simulink library "lib_SecCtrl_MASmsg"  (R2026a)
settings: Solver=VariableStepAuto
undefined symbols (not defined in the file): buses_lf, DiscIntNeverNeededParam, entity, iPs_lf, iQs_lf, last_send, m, Ps_lf, Qs_lf, set_DG_up, set_extra_satur, set_sending_cost, v_buses_mod
libraries: simulink x400, sl_discontinuities x10, eeGeneralControl x5
(part 1 of 12)
settings Model: Creator=atomas  LastModifiedBy=atomas

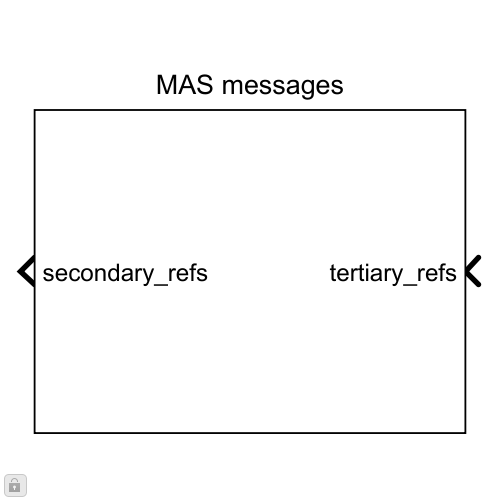
[thumbnail: Simulink's stored preview of the top-level diagram]
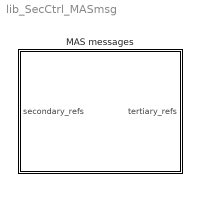
== system lib_SecCtrl_MASmsg ==
  MAS messages : Subsystem  VariantControl=MAS messages

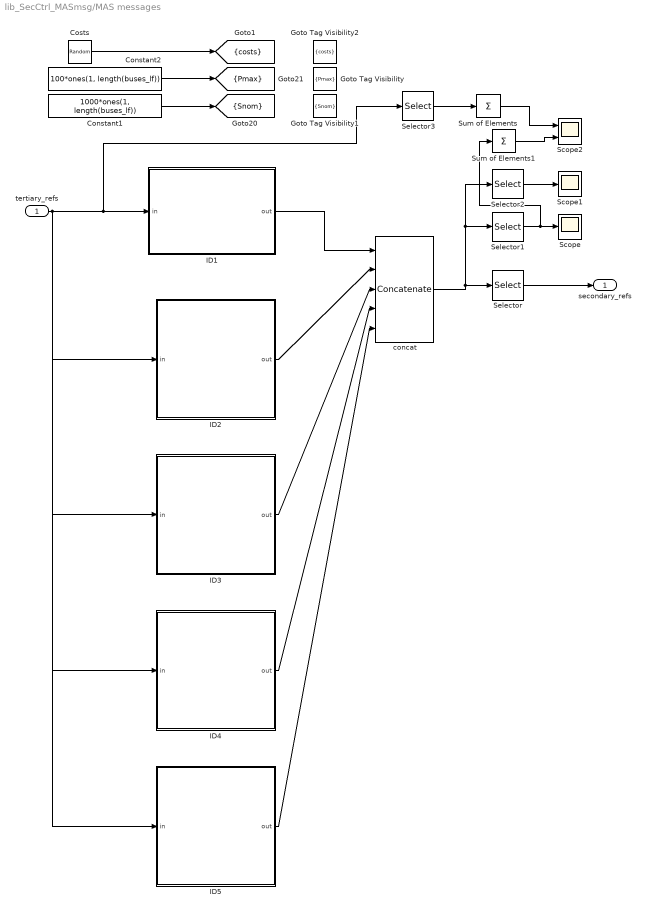
== system lib_SecCtrl_MASmsg/MAS messages ==
  tertiary_refs : Inport
  Constant1 : Constant  Value=1000*ones(1, length(buses_lf))  VectorParams1D=off
  Constant2 : Constant  Value=100*ones(1, length(buses_lf))  VectorParams1D=off
  Costs : RandomNumber  Mean=2*ones(1,length(buses_lf))  Variance=1*ones(1,length(buses_lf))  Seed=1:length(buses_lf)  SampleTime=100  VectorParams1D=off
  Goto Tag Visibility : GotoTagVisibility  GotoTag=Pmax
  Goto Tag Visibility1 : GotoTagVisibility  GotoTag=Snom
  Goto Tag Visibility2 : GotoTagVisibility  GotoTag=costs
  ID1 : Subsystem  VariantControl=multi-agent  mask(gen_agent){ID=1, Leader=Leader, NeighN=2, Neigh1=5, Neigh2=2, Neigh3=0, Neigh4=0, Neigh5=0}
      mask prompts: ID "ID number"; Leader "Leader multi-agent"; NeighN "Number of neighbors"; Neigh1 "Neighbor 1"; Neigh2 "Neighbor 2"; Neigh3 "Neighbor 3"; Neigh4 "Neighbor 4"; Neigh5 "Neighbor 5"
      mask init:
      | block = gcb;
      | NeighN_value = str2double(NeighN);
      | bvarname = get_param(strcat(bdroot, "/", ...
      |     string(extractBetween(gcb, [bdroot '/'], '/'))), 'bvarname');
      | set_param([block '/sentToWorkspace'], 'VariableName', ['sent_' bvarname 'ID' ID])
      | set_param([block '/followingToWorkspace'], 'VariableName', ['following_' bvarname 'ID' ID])
      | set_param([block '/sendingToWorkspace'], 'VariableName', ['sending_' bvarname 'ID' ID])
      | set_param([block '/Receive'], 'MulticastTag', ...
      |     ['ID' ID])
      | set_param([block '/ID'], 'Value', ID)
      | IDnumber = str2double(ID);
      | if strcmp(Leader, "Leader")
      |     set_param([block '/Leader'], 'Value', '1')
      | else
      |     set_param([block '/Leader'], 'Value', '0')
      | end
      | bl_send = find_system(gcb, 'MatchFilter', @Simulink.match.allVariants, 'LookUnderMasks', 'on','MaskType','Send_to_neighbor');
      | 
      | set_param([block '/neigh_left'], 'Value', NeighN)
      | switch NeighN_value % Neighbors
      |     case 1
      |         for i=1:length(bl_send)
      |             set_param(bl_send{i}, 'LabelModeActiveChoice', 'one')
      |             set_param([bl_send{i} '/one/select/Neighbor'], 'const', Neigh1)
      |             set_param([bl_send{i} '/one/Cast'], 'MulticastTag', ['ID' Neigh1])
      |             set_param([bl_send{i} '/one/Castall'], 'MulticastTag', ['ID' Neigh1])
      |         end
      |     case 2
      |         for i=1:length(bl_send)
      |             set_param(bl_send{i}, 'LabelModeActiveChoice', 'two')
      |             set_param([bl_send{i} '/two/select/Neighbor1'], 'const', Neigh1)
      |             set_param([bl_send{i} '/two/Cast1'], 'MulticastTag', ['ID' Neigh1])
      |             set_param([bl_send{i} '/two/Cast1all'], 'MulticastTag', ['ID' Neigh1])
      |             set_param([bl_send{i} '/two/select/Neighbor2'], 'const', Neigh2)
      |             set_param([bl_send{i} '/two/Cast2'], 'MulticastTag', ['ID' Neigh2])
      |             set_param([bl_send{i} '/two/Cast2all'], 'MulticastTag', ['ID' Neigh2])
      |         end
      |     case 3
      |         for i=1:length(bl_send)
      |             set_param(bl_send{i}, 'LabelModeActiveChoice', 'three')
      |             set_param([bl_send{i} '/three/select/Neighbor1'], 'const', Neigh1)
      |             set_param([bl_send{i} '/three/Cast1'], 'MulticastTag', ['ID' Neigh1])
      |             set_param([bl_send{i} '/three/Cast1all'], 'MulticastTag', ['ID' Neigh1])
      |             set_param([bl_send{i} '/three/select/Neighbor2'], 'const', Neigh2)
      |             set_param([bl_send{i} '/three/Cast2'], 'MulticastTag', ['ID' Neigh2])
      |             set_param([bl_send{i} '/three/Cast2all'], 'MulticastTag', ['ID' Neigh2])
      |             set_param([bl_send{i} '/three/select/Neighbor3'], 'const', Neigh3)
      |             set_param([bl_send{i} '/three/Cast3'], 'MulticastTag', ['ID' Neigh3])
      |             set_param([bl_send{i} '/three/Cast3all'], 'MulticastTag', ['ID' Neigh3])
      |         end
      |     case 4
      |         for i=1:length(bl_send)
      |             set_param(bl_send{i}, 'LabelModeActiveChoice', 'four')
      |             set_param([bl_send{i} '/four/select/Neighbor1'], 'const', Neigh1)
      |             set_param([bl_send{i} '/four/Cast1'], 'MulticastTag', ['ID' Neigh1])
      |             set_param([bl_send{i} '/four/Cast1all'], 'MulticastTag', ['ID' Neigh1])
      |             set_param([bl_send{i} '/four/select/Neighbor2'], 'const', Neigh2)
      |             set_param([bl_send{i} '/four/Cast2'], 'MulticastTag', ['ID' Neigh2])
      |             set_param([bl_send{i} '/four/Cast2all'], 'MulticastTag', ['ID' Neigh2])
      |             set_param([bl_send{i} '/four/select/Neighbor3'], 'const', Neigh3)
      |             set_param([bl_send{i} '/four/Cast3'], 'MulticastTag', ['ID' Neigh3])
      |             set_param([bl_send{i} '/four/Cast3all'], 'MulticastTag', ['ID' Neigh3])
      |             set_param([bl_send{i} '/four/select/Neighbor4'], 'const', Neigh4)
      |             set_param([bl_send{i} '/four/Cast4'], 'MulticastTag', ['ID' Neigh4])
      |             set_param([bl_send{i} '/four/Cast4all'], 'MulticastTag', ['ID' Neigh4])
      |         end
      |     case 5
      |         for i=1:length(bl_send)
      |             set_param(bl_send{i}, 'LabelModeActiveChoice', 'five')
      |             set_param([bl_send{i} '/five/select/Neighbor1'], 'const', Neigh1)
      |             set_param([bl_send{i} '/five/Cast1'], 'MulticastTag', ['ID' Neigh1])
      |             set_param([bl_send{i} '/five/Cast1all'], 'MulticastTag', ['ID' Neigh1])
      |             set_param([bl_send{i} '/five/select/Neighbor2'], 'const', Neigh2)
      |             set_param([bl_send{i} '/five/Cast2'], 'MulticastTag', ['ID' Neigh2])
      |             set_param([bl_send{i} '/five/Cast2all'], 'MulticastTag', ['ID' Neigh2])
      |             set_param([bl_send{i} '/five/select/Neighbor3'], 'const', Neigh3)
      |             set_param([bl_send{i} '/five/Cast3'], 'MulticastTag', ['ID' Neigh3])
      |             set_param([bl_send{i} '/five/Cast3all'], 'MulticastTag', ['ID' Neigh3])
      |             set_param([bl_send{i} '/five/select/Neighbor4'], 'const', Neigh4)
      |             set_param([bl_send{i} '/five/Cast4'], 'MulticastTag', ['ID' Neigh4])
      |             set_param([bl_send{i} '/five/Cast4all'], 'MulticastTag', ['ID' Neigh4])
      |             set_param([bl_send{i} '/five/select/Neighbor5'], 'const', Neigh5)
      |             set_param([bl_send{i} '/five/Cast5'], 'MulticastTag', ['ID' Neigh5])
      |             set_param([bl_send{i} '/five/Cast5all'], 'MulticastTag', ['ID' Neigh5])
      |         end
      | end
      mask TypeOptions Leader: No leader | Leader
      mask TypeOptions NeighN: 1 | 2 | 3 | 4 | 5
      mask Callback NeighN:
      | block = gcb;
      | NeighN = str2double(get_param(block, 'NeighN'));
      | param_vis = get_param(block,'MaskVisibilities');
      | block_params = string(fieldnames(get_param(block, 'DialogParameters')));
      | param_vis(find(block_params == 'Neigh1'):find(block_params == 'Neigh5')) = cellstr("on");
      | if NeighN < 5 % Hide some
      |     param_vis(find(block_params == 'Neigh1')+NeighN:find(block_params == 'Neigh5')) = cellstr("off");
      | end
      | set_param(block,'MaskVisibilities',param_vis)
      mask DialogControl Container8 Prompt: Parameters
  ID2 : Subsystem  VariantControl=multi-agent  mask(gen_agent){ID=2, Leader=No leader, NeighN=2, Neigh1=1, Neigh2=3, Neigh3=0, Neigh4=0, Neigh5=0}
      mask prompts: ID "ID number"; Leader "Leader multi-agent"; NeighN "Number of neighbors"; Neigh1 "Neighbor 1"; Neigh2 "Neighbor 2"; Neigh3 "Neighbor 3"; Neigh4 "Neighbor 4"; Neigh5 "Neighbor 5"
      mask init: same as lib_SecCtrl_MASmsg/MAS messages/ID1
      mask TypeOptions Leader: No leader | Leader
      mask TypeOptions NeighN: 1 | 2 | 3 | 4 | 5
      mask Callback NeighN:
      | block = gcb;
      | NeighN = str2double(get_param(block, 'NeighN'));
      | param_vis = get_param(block,'MaskVisibilities');
      | block_params = string(fieldnames(get_param(block, 'DialogParameters')));
      | param_vis(find(block_params == 'Neigh1'):find(block_params == 'Neigh5')) = cellstr("on");
      | if NeighN < 5 % Hide some
      |     param_vis(find(block_params == 'Neigh1')+NeighN:find(block_params == 'Neigh5')) = cellstr("off");
      | end
      | set_param(block,'MaskVisibilities',param_vis)
      mask DialogControl Container8 Prompt: Parameters
  ID3 : Subsystem  VariantControl=multi-agent  mask(gen_agent){ID=3, Leader=No leader, NeighN=2, Neigh1=2, Neigh2=4, Neigh3=0, Neigh4=0, Neigh5=0}
      mask prompts: ID "ID number"; Leader "Leader multi-agent"; NeighN "Number of neighbors"; Neigh1 "Neighbor 1"; Neigh2 "Neighbor 2"; Neigh3 "Neighbor 3"; Neigh4 "Neighbor 4"; Neigh5 "Neighbor 5"
      mask init: same as lib_SecCtrl_MASmsg/MAS messages/ID1
      mask TypeOptions Leader: No leader | Leader
      mask TypeOptions NeighN: 1 | 2 | 3 | 4 | 5
      mask Callback NeighN:
      | block = gcb;
      | NeighN = str2double(get_param(block, 'NeighN'));
      | param_vis = get_param(block,'MaskVisibilities');
      | block_params = string(fieldnames(get_param(block, 'DialogParameters')));
      | param_vis(find(block_params == 'Neigh1'):find(block_params == 'Neigh5')) = cellstr("on");
      | if NeighN < 5 % Hide some
      |     param_vis(find(block_params == 'Neigh1')+NeighN:find(block_params == 'Neigh5')) = cellstr("off");
      | end
      | set_param(block,'MaskVisibilities',param_vis)
      mask DialogControl Container8 Prompt: Parameters
  ID4 : Subsystem  VariantControl=multi-agent  mask(gen_agent){ID=4, Leader=No leader, NeighN=2, Neigh1=3, Neigh2=5, Neigh3=0, Neigh4=0, Neigh5=0}
      mask prompts: ID "ID number"; Leader "Leader multi-agent"; NeighN "Number of neighbors"; Neigh1 "Neighbor 1"; Neigh2 "Neighbor 2"; Neigh3 "Neighbor 3"; Neigh4 "Neighbor 4"; Neigh5 "Neighbor 5"
      mask init: same as lib_SecCtrl_MASmsg/MAS messages/ID1
      mask TypeOptions Leader: No leader | Leader
      mask TypeOptions NeighN: 1 | 2 | 3 | 4 | 5
      mask Callback NeighN:
      | block = gcb;
      | NeighN = str2double(get_param(block, 'NeighN'));
      | param_vis = get_param(block,'MaskVisibilities');
      | block_params = string(fieldnames(get_param(block, 'DialogParameters')));
      | param_vis(find(block_params == 'Neigh1'):find(block_params == 'Neigh5')) = cellstr("on");
      | if NeighN < 5 % Hide some
      |     param_vis(find(block_params == 'Neigh1')+NeighN:find(block_params == 'Neigh5')) = cellstr("off");
      | end
      | set_param(block,'MaskVisibilities',param_vis)
      mask DialogControl Container8 Prompt: Parameters
  ID5 : Subsystem  VariantControl=multi-agent  mask(gen_agent){ID=5, Leader=No leader, NeighN=2, Neigh1=4, Neigh2=1, Neigh3=0, Neigh4=0, Neigh5=0}
      mask prompts: ID "ID number"; Leader "Leader multi-agent"; NeighN "Number of neighbors"; Neigh1 "Neighbor 1"; Neigh2 "Neighbor 2"; Neigh3 "Neighbor 3"; Neigh4 "Neighbor 4"; Neigh5 "Neighbor 5"
      mask init: same as lib_SecCtrl_MASmsg/MAS messages/ID1
      mask TypeOptions Leader: No leader | Leader
      mask TypeOptions NeighN: 1 | 2 | 3 | 4 | 5
      mask Callback NeighN:
      | block = gcb;
      | NeighN = str2double(get_param(block, 'NeighN'));
      | param_vis = get_param(block,'MaskVisibilities');
      | block_params = string(fieldnames(get_param(block, 'DialogParameters')));
      | param_vis(find(block_params == 'Neigh1'):find(block_params == 'Neigh5')) = cellstr("on");
      | if NeighN < 5 % Hide some
      |     param_vis(find(block_params == 'Neigh1')+NeighN:find(block_params == 'Neigh5')) = cellstr("off");
      | end
      | set_param(block,'MaskVisibilities',param_vis)
      mask DialogControl Container8 Prompt: Parameters
  Scope : Scope
      settings: ActiveDisplayYMinimum=3.7204  ActiveDisplayYMaximum=6.2533  DataLoggingVariableName=ScopeData2
  Scope1 : Scope
      settings: ActiveDisplayYMinimum=0.24945  ActiveDisplayYMaximum=4.0188
  Scope2 : Scope  NumInputPorts=2
      settings: ActiveDisplayYMinimum=9.9395  ActiveDisplayYMaximum=10.281  DataLoggingVariableName=ScopeData3
  Selector : Selector  NumberOfDimensions=2  InputPortWidth=3  IndexOptions=Index vector (dialog),Select all  Indices=1:6,1  OutputSizes=1,1
  Selector1 : Selector  NumberOfDimensions=2  InputPortWidth=3  IndexOptions=Index vector (dialog),Select all  Indices=7,1  OutputSizes=1,1
  Selector2 : Selector  NumberOfDimensions=2  InputPortWidth=3  IndexOptions=Index vector (dialog),Select all  Indices=8,1  OutputSizes=1,1
  Selector3 : Selector  NumberOfDimensions=2  InputPortWidth=3  IndexOptions=Index vector (dialog),Select all  Indices=2,1  OutputSizes=1,1
  Sum of Elements : Sum  Inputs=+
  Sum of Elements1 : Sum  Inputs=+
  concat : Concatenate  NumInputs=length(buses_lf)  Mode=Multidimensional array  ConcatenateDimension=2
  secondary_refs : Outport
  tag scope: Pmax=scoped, Snom=scoped, costs=scoped
  wires:
  ID5/1(out) -> concat/5
  ID4/1(out) -> concat/4
  ID3/1(out) -> concat/3
  ID2/1(out) -> concat/2
  Costs/1 -> [costs]
  Sum of Elements1/1 -> Scope2/2
  Sum of Elements/1 -> Scope2/1
  Selector3/1 -> Sum of Elements/1
  Selector2/1 -> Scope1/1
  Selector1/1 -> Scope/1, Sum of Elements1/1
  Selector/1 -> secondary_refs/1
  ID1/1(out) -> concat/1
  Constant1/1 -> [Snom]
  Constant2/1 -> [Pmax]
  tertiary_refs/1 -> ID5/1(in), ID4/1(in), ID3/1(in), ID2/1(in), ID1/1(in), Selector3/1
  concat/1 -> Selector/1, Selector1/1, Selector2/1
